simulink model "hardwareModel_6"  (R2026a)
settings: Solver=FixedStepAuto  StopTime=inf  EnableMultiTasking=on
values from neighbouring files (symbols this model uses):
  Ts = 0.01    [modelParameters.m]
libraries: arduinomotorcarrierlib x3, simulink x1, eeGeneralControl x1, arduinosensorlib x1
settings Model: SILPILModeSetting=veronly  ExtModeTrigDuration=2  Creator=bkhusain  LastModifiedBy=paolo
settings OptimizationCC: PassReuseOutputArgsThreshold=0.0
settings HardwareCC: ProdLargestAtomicInteger=Long  ProdLargestAtomicFloat=Double  ProdHWDeviceType=ARM Compatible->ARM Cortex  UseEmbeddedCoderFeatures=off  UseSimulinkCoderFeatures=off
settings RTWCC: SystemTargetFile=ert.tlc  HardwareBoard=Arduino Nano 33 IoT  TLCOptions=-aInlineSetEventsForThisBaseRateFcn=TLC_FALSE -aSuppressMultiTaskScheduler=TLC_FALSE -aRateBasedStepFcn=1  Toolchain=Arduino ARM  BuildConfiguration=Faster Runs  Description=Embedded Coder
settings ERTTargetCC: ExtModeTransport=2.0  ExtModeStaticAllocSize=8192.0  DynamicArrayContainerType=coder::array  ERTCustomFileBanners=off  SupportContinuousTime=on  SupportNonInlinedSFcns=on  SupportVariableSizeSignals=on  ModelStepFunctionPrototypeControlCompliant=off
settings SimscapeCC: SimscapeNominalValues="[{\"value\":\"1\",\"unit\":\"A\"},{\"value\":\"1\",\"unit\":\"bar\"},{\"value\":\"1\",\"unit\":\"cm^2\"},{\"value\":\"1\",\"unit\":\"cm^3/s\"},{\"value\":\"1\",\"unit\":\"kJ/kg\"},{\"value\":\"1\",\"unit\":\"kW\"},{\"value\":\"1\",\"unit\":\"l\"},{\"value\":\"1\",\"unit\":\"N\"},{\"value\":\"1\",\"unit\":\"N*m\"},{\"value\":\"1\",\"unit\":\"V\"}]"  SimscapeLogType=none  SimscapeLogDataHistory=5000.0

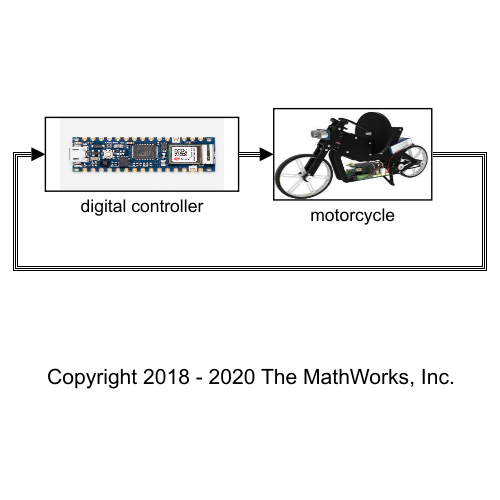
[thumbnail: Simulink's stored preview of the top-level diagram]
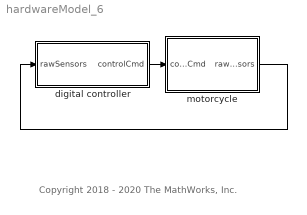
== system hardwareModel_6 ==
  note: Copyright 2018 - 2020 The MathWorks, Inc.
  digital controller : Subsystem
      mask Display: image('$imagefile'); % Use "Edit Image" on toolstrip to change.
  motorcycle : Subsystem
      mask Display: image('$imagefile'); % Use "Edit Image" on toolstrip to change.
  wires:
  digital controller/1(controlCmd) -> motorcycle/1(controlCmd)
  motorcycle/1(rawSensors) -> digital controller/1(rawSensors)

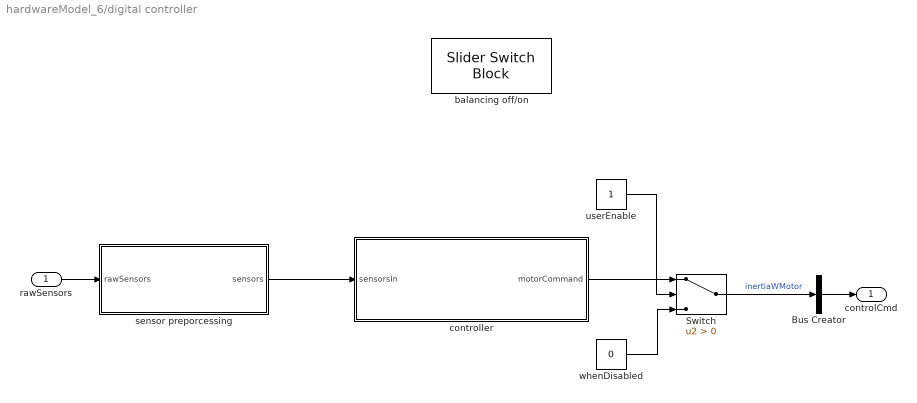
== system hardwareModel_6/digital controller ==
  rawSensors : Inport
  Bus Creator : BusCreator  Inputs=1
  Switch : Switch  Criteria=u2 > Threshold  SaturateOnIntegerOverflow=off  InputSameDT=off
  balancing off/on : SliderSwitchBlock  LabelPosition=Hide
  controller : Subsystem
  sensor preporcessing : Subsystem
  userEnable : Constant  SampleTime=Ts
  whenDisabled : Constant  Value=0  SampleTime=Ts
  controlCmd : Outport
  wires:
  Bus Creator/1 -> controlCmd/1
  rawSensors/1 -> sensor preporcessing/1(rawSensors)
  sensor preporcessing/1(sensors) -> controller/1(sensorsIn)
  whenDisabled/1 -> Switch/3
  controller/1(motorCommand) -> Switch/1
  Switch/1 -> Bus Creator/1  "inertiaWMotor"
  userEnable/1 -> Switch/2

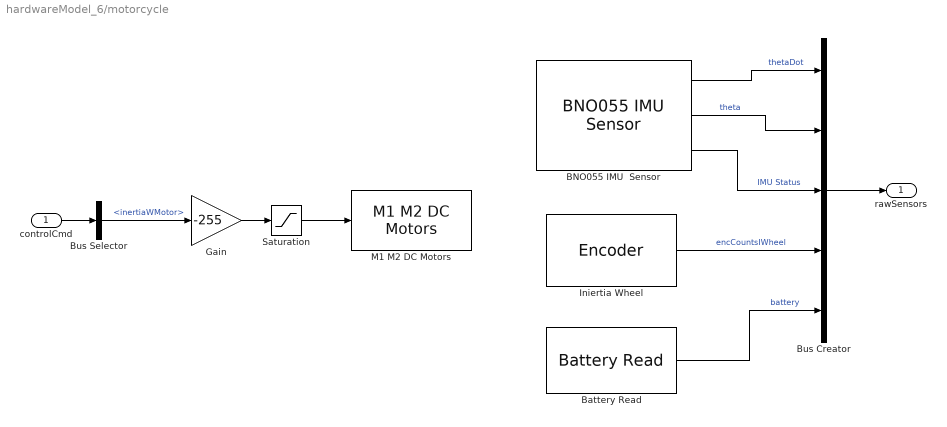
== system hardwareModel_6/motorcycle ==
  controlCmd : Inport
  BNO055 IMU  Sensor : arduinosensorlib/BNO055 IMU Sensor  I2CModule=0  SlaveAddress=0x28  OperationMode=Fusion  Accel=off  AngularRate=on  MagField=off  EulerAngles=on  Quat=off  LinearAccel=off  GravityVector=off  Status=on  Timestamp=off  AccelRange=4G  AccelBW=62.5 Hz  GyroRange=2000 dps  GyroBW=32 Hz  MagODR=10 Hz  spf=1  SampleTime=Ts  blockPlatform=ARDUINO  QueueSizeFactor=1
  Battery Read : arduinomotorcarrierlib/Battery Read  SlaveAddress=uint8( hex2dec( '66' ) )  blockPlatform=ARDUINO  SampleTime=Ts
  Bus Creator : BusCreator  Inputs=5
  Bus Selector : BusSelector  OutputSignals=inertiaWMotor
  Gain : Gain  Gain=-255
  Iniertia Wheel : arduinomotorcarrierlib/Encoder  SlaveAddress=uint8( hex2dec( '66' ) )  blockPlatform=ARDUINO  Encoder=1  ShowSpeed=off  ResetOption=on  SampleTime=Ts
  M1 M2 DC Motors : arduinomotorcarrierlib/M1 M2 DC Motors  SlaveAddress=uint8( hex2dec( '66' ) )  blockPlatform=ARDUINO  MotorNumber=M1  MotorCarrierPWMFreq=100
  Saturation : Saturate  UpperLimit=255  LowerLimit=-255
  rawSensors : Outport
  wires:
  BNO055 IMU  Sensor/1 -> Bus Creator/1  "thetaDot"
  BNO055 IMU  Sensor/2 -> Bus Creator/2  "theta"
  BNO055 IMU  Sensor/3 -> Bus Creator/3  "IMU Status"
  Iniertia Wheel/1 -> Bus Creator/4  "encCountsIWheel"
  Battery Read/1 -> Bus Creator/5  "battery"
  Bus Creator/1 -> rawSensors/1
  controlCmd/1 -> Bus Selector/1
  Gain/1 -> Saturation/1
  Bus Selector/1 -> Gain/1  "<inertiaWMotor>"
  Saturation/1 -> M1 M2 DC Motors/1

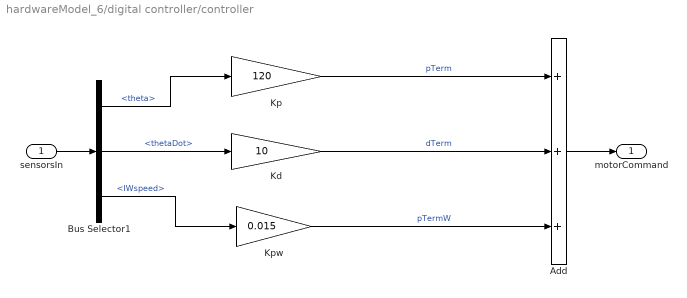
== system hardwareModel_6/digital controller/controller ==
  sensorsIn : Inport
  Add : Sum  Inputs=+++
  Bus Selector1 : BusSelector  OutputSignals=theta,thetaDot,IWspeed
  Kd : Gain  Gain=10
  Kp : Gain  Gain=120
  Kpw : Gain  Gain=0.015
  motorCommand : Outport
  wires:
  Bus Selector1/3 -> Kpw/1  "<IWspeed>"
  Kpw/1 -> Add/3  "pTermW"
  Kd/1 -> Add/2  "dTerm"
  Bus Selector1/2 -> Kd/1  "<thetaDot>"
  Bus Selector1/1 -> Kp/1  "<theta>"
  Kp/1 -> Add/1  "pTerm"
  sensorsIn/1 -> Bus Selector1/1
  Add/1 -> motorCommand/1

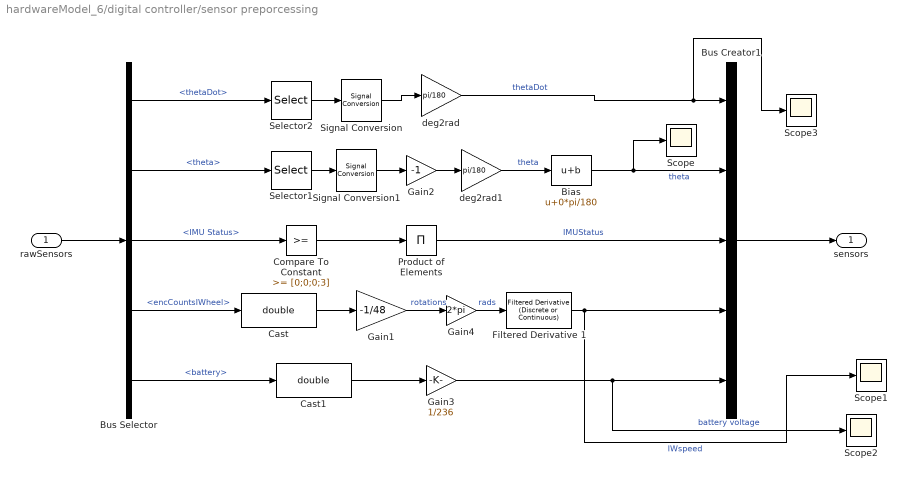
== system hardwareModel_6/digital controller/sensor preporcessing ==
  rawSensors : Inport
  Bias : Bias  Bias=0*pi/180  SaturateOnIntegerOverflow=off
  Bus Creator1 : BusCreator  Inputs=5
  Bus Selector : BusSelector  OutputSignals=thetaDot,theta,IMU Status,encCountsIWheel,battery
  Cast : DataTypeConversion  OutDataTypeStr=double  SaturateOnIntegerOverflow=off  RndMeth=Floor
  Cast1 : DataTypeConversion  OutDataTypeStr=double  SaturateOnIntegerOverflow=off  RndMeth=Floor
  Compare To Constant : simulink/Logic and Bit Operations/Compare To Constant  relop=>=  const=[0;0;0;3]  OutDataTypeStr=boolean
  Filtered Derivative 1 : eeGeneralControl/Filtered Derivative (Discrete or Continuous)  K=1  T=0.1  B=inf  A=-inf  minRatio=10  init_option=Inherited from block input  x0=0  Ts=Ts
  Gain1 : Gain  Gain=-1/48
  Gain2 : Gain  Gain=-1
  Gain3 : Gain  Gain=1/236
  Gain4 : Gain  Gain=2*pi
  Product of Elements : Product  Inputs=*
  Scope{,1..3} (4 alike) : Scope
      Scope settings: ActiveDisplayYMinimum=0.048814677516716413  ActiveDisplayYMaximum=0.29152452662217787
      Scope1 settings: ActiveDisplayYMinimum=-421.30755284787938  ActiveDisplayYMaximum=-167.75380895923718  DataLoggingVariableName=ScopeData2
      Scope2 settings: ActiveDisplayYMinimum=3.6541313559322033  ActiveDisplayYMaximum=3.6806144067796609  DataLoggingVariableName=ScopeData3
      Scope3 settings: ActiveDisplayYMinimum=-1.5207544646478715  ActiveDisplayYMaximum=1.2949524926711051  DataLoggingVariableName=ScopeData4
  Selector1 : Selector  InputPortWidth=3  IndexOptions=Index vector (dialog)  Indices=[2]  OutputSizes=1
  Selector2 : Selector  InputPortWidth=3  IndexOptions=Index vector (dialog)  Indices=[2]  OutputSizes=1
  Signal Conversion : SignalConversion  OverrideOpt=off
  Signal Conversion1 : SignalConversion  OverrideOpt=off
  deg2rad : Gain  Gain=pi/180
  deg2rad1 : Gain  Gain=pi/180
  sensors : Outport
  wires:
  Bus Selector/4 -> Cast/1  "<encCountsIWheel>"
  Compare To Constant/1 -> Product of Elements/1
  Bus Selector/5 -> Cast1/1  "<battery>"
  Selector2/1 -> Signal Conversion/1
  Bus Selector/2 -> Selector1/1  "<theta>"
  Selector1/1 -> Signal Conversion1/1
  Cast1/1 -> Gain3/1
  Bus Selector/3 -> Compare To Constant/1  "<IMU Status>"
  rawSensors/1 -> Bus Selector/1
  Product of Elements/1 -> Bus Creator1/3  "IMUStatus"
  Filtered Derivative 1/1 -> Scope1/1, Bus Creator1/4  "IWspeed"
  deg2rad1/1 -> Bias/1  "theta"
  Bus Selector/1 -> Selector2/1  "<thetaDot>"
  Gain3/1 -> Scope2/1, Bus Creator1/5  "battery voltage"
  Bus Creator1/1 -> sensors/1
  Signal Conversion1/1 -> Gain2/1
  Gain2/1 -> deg2rad1/1
  Signal Conversion/1 -> deg2rad/1
  Cast/1 -> Gain1/1
  Gain1/1 -> Gain4/1  "rotations"
  Gain4/1 -> Filtered Derivative 1/1  "rads"
  deg2rad/1 -> Scope3/1, Bus Creator1/1  "thetaDot"
  Bias/1 -> Scope/1, Bus Creator1/2  "theta"
